simulink subsystem "Leg_Force_Unwired"  (R2026a)
settings: Solver=VariableStepAuto
settings Model: Creator=asing  LastModifiedBy=asing

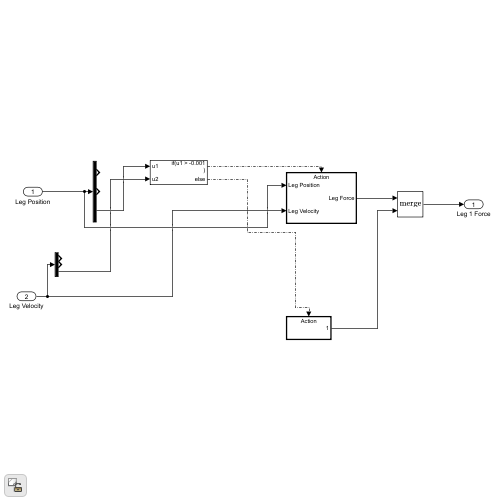
[thumbnail: Simulink's stored preview of the top-level diagram]
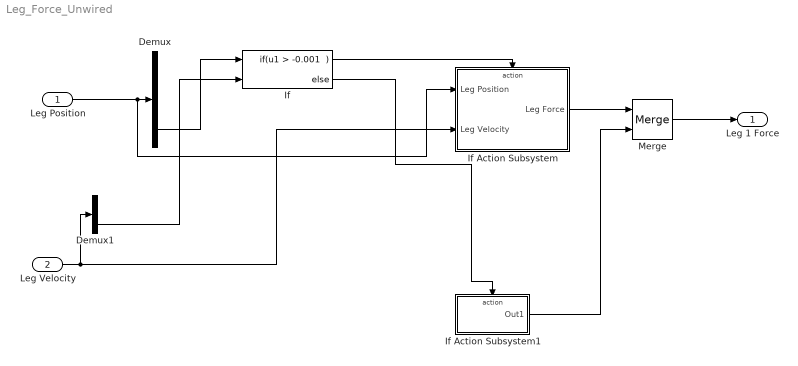
== system Leg_Force_Unwired ==
  Leg Position : Inport
  Leg Velocity : Inport  Port=2
  Demux : Demux  Outputs=3
  Demux1 : Demux  Outputs=3
  If : If  NumInputs=2  IfExpression=u1 > -0.001
  If Action Subsystem : Subsystem  TreatAsAtomicUnit=on
  If Action Subsystem1 : Subsystem  TreatAsAtomicUnit=on
  Merge : Merge
  Leg 1 Force : Outport
  wires:
  Leg Position/1 -> Demux/1, If Action Subsystem/1(Leg Position)
  If/2 -> If Action Subsystem1/Action
  If Action Subsystem/1(Leg Force) -> Merge/1
  If Action Subsystem1/1(Out1) -> Merge/2
  Merge/1 -> Leg 1 Force/1
  Leg Velocity/1 -> If Action Subsystem/2(Leg Velocity), Demux1/1
  If/1 -> If Action Subsystem/Action
  Demux/3 -> If/1
  Demux1/3 -> If/2

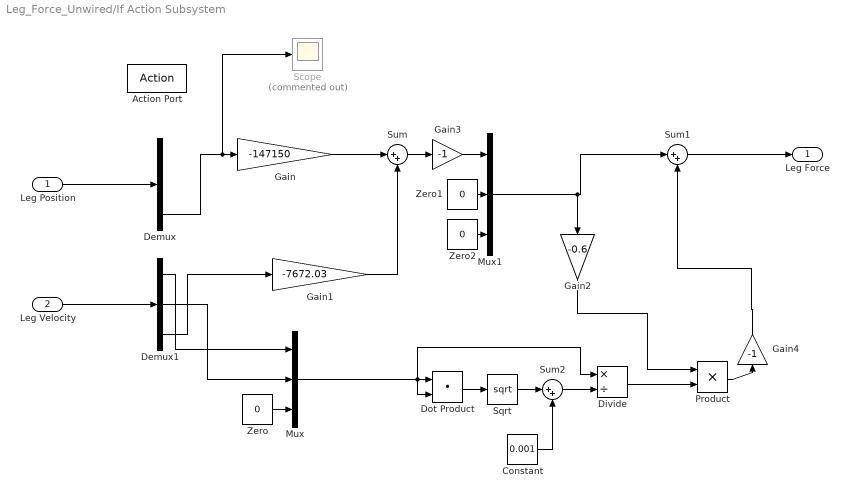
== system Leg_Force_Unwired/If Action Subsystem ==
  Leg Position : Inport
  Leg Velocity : Inport  Port=2
  Action Port : ActionPort
  Constant : Constant  Value=0.001
  Demux : Demux  Outputs=3
  Demux1 : Demux  Outputs=3
  Divide : Product  Inputs=*/
  Dot Product : DotProduct  OutDataTypeStr=Inherit: Inherit via internal rule
  Gain : Gain  Gain=-147150
  Gain1 : Gain  Gain=-7672.03
  Gain2 : Gain  Gain=-0.6
  Gain3 : Gain  Gain=-1
  Gain4 : Gain  Gain=-1
  Mux : Mux  Inputs=3
  Mux1 : Mux  Inputs=3
  Product : Product
  Scope : Scope  Commented=on
      settings: ActiveDisplayYMinimum=-1  ActiveDisplayYMaximum=1  DataLoggingVariableName=ScopeData69
  Sqrt : Sqrt
  Sum : Sum  Inputs=|++
  Sum1 : Sum  Inputs=|++
  Sum2 : Sum  Inputs=|++
  Zero : Constant  Value=0  OutDataTypeStr=Inherit: Inherit via back propagation
  Zero1 : Constant  Value=0  OutDataTypeStr=Inherit: Inherit via back propagation
  Zero2 : Constant  Value=0  OutDataTypeStr=Inherit: Inherit via back propagation
  Leg Force : Outport
  wires:
  Gain4/1 -> Sum1/2
  Gain3/1 -> Mux1/1
  Zero/1 -> Mux/3
  Demux/3 -> Gain/1, Scope/1
  Mux1/1 -> Gain2/1, Sum1/1
  Zero2/1 -> Mux1/3
  Zero1/1 -> Mux1/2
  Sum/1 -> Gain3/1
  Constant/1 -> Sum2/2
  Sum2/1 -> Divide/2
  Sqrt/1 -> Sum2/1
  Sum1/1 -> Leg Force/1
  Product/1 -> Gain4/1
  Gain2/1 -> Product/1
  Divide/1 -> Product/2
  Dot Product/1 -> Sqrt/1
  Mux/1 -> Divide/1, Dot Product/1, Dot Product/2
  Demux1/1 -> Mux/1
  Demux1/2 -> Mux/2
  Demux1/3 -> Gain1/1
  Gain1/1 -> Sum/2
  Gain/1 -> Sum/1
  Leg Velocity/1 -> Demux1/1
  Leg Position/1 -> Demux/1

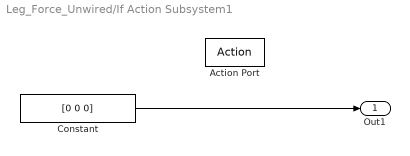
== system Leg_Force_Unwired/If Action Subsystem1 ==
  Action Port : ActionPort
  Constant : Constant  Value=[0 0 0]
  Out1 : Outport
  wires:
  Constant/1 -> Out1/1
